simulink subsystem "pendulum_linear"  (R2024b)
settings: Solver=VariableStepAuto  StartTime=0.0  StopTime=10.0  RelTol=1e-3
undefined symbols (not defined in the file): params, plant_ss
settings Model: Creator=dsagn  LastModifiedBy=dsagn
settings ModelReferenceCC: UpdateModelReferenceTargets=IfOutOfDate
settings SFSimCC: SimGPUStackLimitPerThread=51200
settings RTWCC: GPUStackLimitPerThread=51200  GPUComputeCapability=7.5
settings ConfigComp: CovMetricSettings=de  CovBoundaryAbsTol=1.0e-5

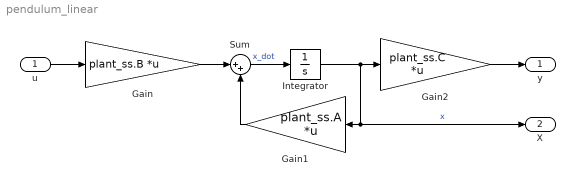
== system pendulum_linear ==
  u : Inport
  Gain : Gain  Gain=plant_ss.B  Multiplication=Matrix(K*u) (u vector)
  Gain1 : Gain  Gain=plant_ss.A  Multiplication=Matrix(K*u) (u vector)
  Gain2 : Gain  Gain=plant_ss.C  Multiplication=Matrix(K*u) (u vector)
  Integrator : Integrator  InitialCondition=params.IC
  Sum : Sum  Inputs=|++
  y : Outport  VectorParamsAs1DForOutWhenUnconnected=off
  X : Outport  Port=2
  wires:
  u/1 -> Gain/1
  Integrator/1 -> Gain1/1, X/1, Gain2/1  "x"
  Gain1/1 -> Sum/2
  Gain/1 -> Sum/1
  Gain2/1 -> y/1
  Sum/1 -> Integrator/1  "x_dot"
